simulink model "all_nn_0001_0127"  (R2026a)
settings: Solver=ode45  StopTime=40  AbsTol=1e-6
undefined symbols (not defined in the file): u_ts
settings Model: ExtModeTrigMode=oneshot  ExtModeArmWhenConnect=off  TunableVars=prueba  TunableVarsStorageClass=Auto  Creator=The MathWorks Inc.  LastModifiedBy=harry_31916
settings DataIOCC: SignalLoggingName=sigsOut
settings OptimizationCC: BooleanDataType=off  InitFltsAndDblsToZero=on
settings DebuggingCC: SaveWithParameterizedLinksMsg=none  UnderspecifiedInitializationDetection=Classic  SignalResolutionControl=TryResolveAllWithWarning  MultiTaskDSMMsg=warning  MultiTaskCondExecSysMsg=none
settings HardwareCC: ProdHWDeviceType=32-bit Generic  TargetUnknown=on
settings RTWCC: TemplateMakefile=grt_vc.tmf
settings GRTTargetCC: TargetFcnLib=ansi_tfl_tmw.mat  CombineOutputUpdateFcns=off  GRTInterface=on

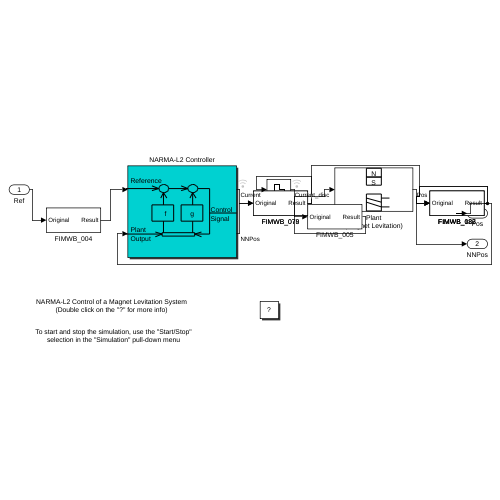
[thumbnail: Simulink's stored preview of the top-level diagram]
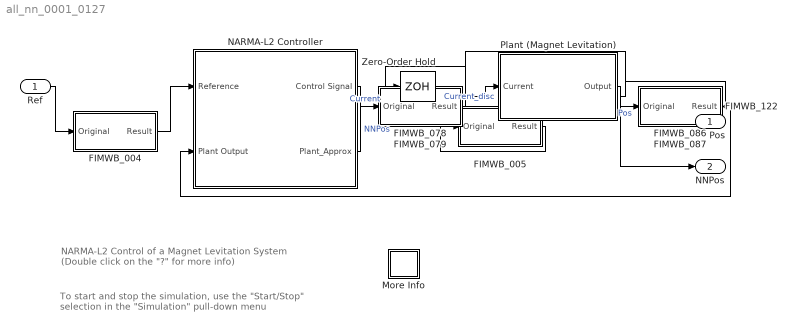
== system all_nn_0001_0127 ==
  note: NARMA-L2 Control of a Magnet Levitation System
      | (Double click on the "?" for more info)
  note: To start and stop the simulation, use the "Start/Stop"
      | selection in the "Simulation" pull-down menu
  Ref : Inport  Interpolate=off
  FIMWB_004 : Subsystem  Tag=fimwb.fault.4
  FIMWB_005 : Subsystem  Tag=fimwb.fault.5
  FIMWB_078 : Subsystem  Tag=fimwb.fault.78
  FIMWB_079 : Subsystem  Tag=fimwb.fault.79
  FIMWB_086 : Subsystem  Tag=fimwb.fault.86
  FIMWB_087 : Subsystem  Tag=fimwb.fault.87
  FIMWB_122 : Subsystem  Tag=fimwb.fault.122
  More Info : Subsystem
      mask Display: disp('?')
  NARMA-L2 Controller : Subsystem  mask(NARMA-L2 Controller){Ts=0.01, S1=9, Ni=3, Nj=2, sim_file=ballrepel0, trainfun=trainlm, Use_validation=1, Use_Testing=1, max_i=4, min_i=-1, max_i_int=1, min_i_int=0.1, sam_training=10000, epochs=100, minp=-0.97682887932966278033, maxp=3.9954019738068033973, mint=0.0012713472471279200528, maxt=3.9954019738068033973, Normalize=1, IW1_1=[2.8569160539166240653 3.855137973617931646 2.4478436741338867044 0.86889986713150191289;0.86019748624118552716 -0.76099748761653862594 0.12978383283599650988 -0.032681949683702651854;-0.61268951567451579443 -1.3546538767805089698 -1.0357145918607806312 -2.2450213565212968625;-0.61363639390594604262 3.6302797918127760468 -2.9742392265006136753 3.7505205510025696469;8.2159425419552984948 -0.34781842703357196411 -0.63990978222347083548 3.2203753164455033442;-0.55585558555235048406 1.7347260034225613357 -0.48782067399191109125 0.15519292550861990554;0.14490936608588075862 0.091344996887225110571 -1.9999177921909609967 -1.7398058021589537514;-0.011364174849476511159 0.17210174153872684344 -0.063003341331735851494 0.016356680939399299846;1.9115353490253352842 -1.6928290742800000679 0.26139115964517828372 -0.083521590880859600259], IW3_2=[2.094012153469472004 4.1391617494602943594 0.46017743638858904509 1.4212453617040687881;-0.8698291152927356551 -0.91216393263270156844 -1.7725276755524563832 -1.8256681774546807961;-1.5212626080129232342 -1.9638393468584769419 -0.13083206166844379981 0.69514443101461376173;1.1067100747068669975 1.1077222299712199405 -1.6499992245985941608 -0.10283142888325141895;1.7627456897433946281 0.12387727106338465577 -0.74345872574560734058 1.3295242695796243293;1.3902623706994512442 1.2486843128494045096 0.60100357220348832321 1.8703374952532536568;-1.2652620294004319756 -0.81003971518970829813 0.35904126229892613376 -2.3590512744589045013;-1.7962091138833455872 0.33004248956449860897 1.1996735804361835509 -0.75846441756669458201;1.6085665816521634852 -0.65960011993077061199 2.0409314507416924656 1.300834198719902135], IW5_3=-0.86130216008060445088, LW2_1=[5.755548244449743792e-05 2.1941017287714528194 -0.00044492281828180146918 -0.00039237971120205448854 1.8234323877817898572e-06 0.042708432151687514278 0.00025330049100551882673 4.7927194580095164866 0.41991364122019325666], LW4_3=[1.1796229157074380467 1.4349048600431937306 -0.8972572979998952869 -2.3386270416842869224 -0.096692942439327439486 -0.63438599215078772531 -2.7379194644695021843 3.0145214892072624835 2.1741978843496214679], LW5_4=0.59967978592905768487, LW6_5=0.00041169382628446888304, LW6_2=0.99216750753278892816, B1=[-2.0540485030510766684;-0.2820456548276839559;-1.4224984046874724619;0.011980000365264734455;-3.2833055176157808219;1.1020848049883287256;2.2616940700361274352;-0.14165422591960777354;1.0889769241125049071], B2=0.90790507647934137747, B3=[-0.99822473976112757743;-1.1258457923320430716;1.0030562696131117839;3.6020655513043440266;-0.0251859643674823587;1.2763936285299730677;-2.2740100652873409537;-3.0720977283302817185;1.7835104510380932474], B4=0.8636776698074994929, Limit_output=1, min_output=0, max_output=Inf, Use_Previous_Weights=1}
      mask prompts: Ts "Sample time"; trainfun "Training function"
      mask help: NARMA-L2 Controller. You first train a neural network model of the plant to be controlled. The controller is a rearrangement of the trained plant model. Double-click the NARMA-L2 Controller block to begin the plant training.
      mask init:
      | xl = [0    .4   NaN  .33  .55   .55  .33  .33  NaN .80  .92 .92];
      | yl = [.95 .95 NaN  .75  .75   .55  .55  .75  NaN  .95 .95 .65];
      | x2 = [0    .43 NaN .45 .45    NaN .92 1.2 NaN .63 .85 .85 .63 .63 ];
      | y2 = [.39 .39 NaN  .41 .55   NaN .65 .65 NaN .75 .75  .55  .55  .75];
      | x3 = [.45 .45 NaN .42 .45 .48  NaN .33 .4 .33];
      | y3 = [.75 .90 NaN .83 .90 .83  NaN  .98 .95 .92];
      | x4 = [.75 .75 NaN .72 .75 .78  NaN  .5 .7 NaN .63 .7 .63];
      | y4 = [.75 .90 NaN .83 .90 .83  NaN .95 .95 NaN .98 .95 .92];
      | x5 = [.43 .43 .77 .77 .43 NaN .36 .43 .36 NaN .75 .75];
      | y5 = [.37 .41 .41 .37 .37 NaN .42 .39 .36 NaN .41 .55];
      | x6 = [.92 .92 .77 NaN .84 .77 .84];
      | y6 = [.65 .39 .39 NaN .42 .39 .36];
      | x1t=.03; y1t=.31;
      | x2t=.03; y2t=.85;
      | x8t=.03;y8t=.21;
      | x3t=.77; y3t=.53;
      | x4t=.77; y4t=.44;
      | x5t=.34; y5t=.49;
      | x6t=.58; y6t=.49;
      | 
      | 
      | t=(0:24)/24*2*pi;
      | xs = .05*cos(t);
      | ys = .05*sin(t);
      | xs1=xs+.45;
      | ys1=ys+.95;
      | xs2=xs+.75;
      | ys2=ys+.95;
      settings: OpenFcn=nncontrolutil('nnident','',gcbh,gcb,'narma_l2');
      mask TypeOptions trainfun: trainbfg | trainbr  | traincgb | traincgf | traincgp | traingd | traingdm | traingda | traingdx | trainlm  | trainoss | trainrp  | trainscg
      mask Display:
      | plot([[xl NaN x2]*.9-.075 ], [[yl  NaN y2]*.9-.1 ]);
      | plot([[x3 NaN xs1 NaN xs2]*.9-.075 ], [[y3 NaN ys1 NaN ys2]*.9-.1 ]);
      | plot([x4 NaN x5]*.9-.075,[y4 NaN y5]*.9-.1);
      | plot([x6 NaN ]*.9-.075,[y6 NaN ]*.9-.1);
      | text(x1t,y1t,'Plant');
      | text(x8t,y8t,'Output');
      | text(x2t,y2t,'Reference');
      | text(x3t,y3t,'Control');
      | text(x4t,y4t,'Signal');
      | text(x5t,y5t,'f');
      | text(x6t,y6t,'g');
  Plant (Magnet Levitation) : Subsystem
      mask init:
      | x1=[-2 -2 2 2 -2 NaN -2 -2 2 2 -2];
      | y1=[5 4 4 5 5 NaN 2 0 0 2 2];
      | x2=[-2 -2 2 2 -2 NaN -2   2  NaN -2 2 NaN 2    4    NaN 2  4];
      | y2=[4  3  3 4  4 NaN 1.5 1  NaN 1 .5 NaN 1.5 1.5 NaN .5 .5];
      | x1t = -.5 ; y1t = 4.4;
      | x2t = -.5; y2t = 3.4;
      mask Display:
      | plot([-10],[0],[10],[5]);
      | plot([x1 NaN x2],[y1 NaN y2]);
      | text(x1t,y1t,'N')
      | text(x2t,y2t,'S')
  Zero-Order Hold : ZeroOrderHold  SampleTime=u_ts
  Pos : Outport  VectorParamsAs1DForOutWhenUnconnected=off
  NNPos : Outport  Port=2  VectorParamsAs1DForOutWhenUnconnected=off
  wires:
  Plant (Magnet Levitation)/1(Output) -> FIMWB_122/1(Original)  "Pos"
  FIMWB_122/1(Result) -> FIMWB_086/1(Original), FIMWB_087/1(Original)
  Ref/1 -> FIMWB_004/1(Original)
  FIMWB_004/1(Result) -> NARMA-L2 Controller/1(Reference)
  Zero-Order Hold/1 -> FIMWB_005/1(Original)  "Current_disc"
  FIMWB_005/1(Result) -> Plant (Magnet Levitation)/1(Current)
  NARMA-L2 Controller/1(Control Signal) -> FIMWB_078/1(Original)  "Current"
  FIMWB_078/1(Result) -> Zero-Order Hold/1
  NARMA-L2 Controller/2(Plant_Approx) -> FIMWB_079/1(Original)  "NNPos"
  FIMWB_079/1(Result) -> NNPos/1
  FIMWB_086/1(Result) -> Pos/1
  FIMWB_087/1(Result) -> NARMA-L2 Controller/2(Plant Output)

== system all_nn_0001_0127/FIMWB_004 ==
  Original : Inport
  Result : Outport
  wires:
  Original/1 -> Result/1

== system all_nn_0001_0127/FIMWB_005 ==
  Original : Inport
  Result : Outport
  wires:
  Original/1 -> Result/1

== system all_nn_0001_0127/FIMWB_078 ==
  Original : Inport
  Result : Outport
  wires:
  Original/1 -> Result/1

== system all_nn_0001_0127/FIMWB_079 ==
  Original : Inport
  Result : Outport
  wires:
  Original/1 -> Result/1

== system all_nn_0001_0127/FIMWB_086 ==
  Original : Inport
  Result : Outport
  wires:
  Original/1 -> Result/1

== system all_nn_0001_0127/FIMWB_087 ==
  Original : Inport
  Result : Outport
  wires:
  Original/1 -> Result/1

== system all_nn_0001_0127/FIMWB_122 ==
  Original : Inport
  Result : Outport
  wires:
  Original/1 -> Result/1

== system all_nn_0001_0127/More Info ==
  note: This system simulates NARMA-L2 control
      | of a magnet suspended by an electromagnet.
  note: Double-click on the NARMA-L2 Controller block
      | to train the neural network controller and plant model.
  note: For more information on what the controller
      | does, look under the mask of the NARMA-L2
      | Controller block.

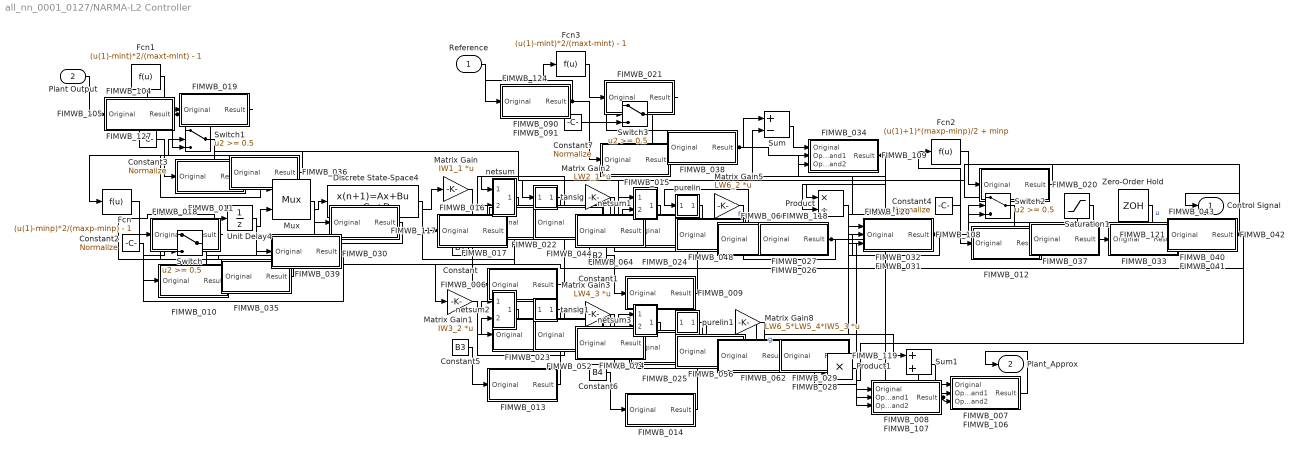
== system all_nn_0001_0127/NARMA-L2 Controller ==
  Reference : Inport
  Plant Output : Inport  Port=2
  Constant : Constant  Value=B1
  Constant1 : Constant  Value=B2
  Constant{2..4,7} (4 alike) : Constant  Value=Normalize
  Constant5 : Constant  Value=B3
  Constant6 : Constant  Value=B4
  Discrete State-Space4 : DiscreteStateSpace  A=blkdiag([zeros(1,Nj-1);eye(Nj-2,Nj-2) zeros(Nj-2,1)],[zeros(1,Ni-1);eye(Ni-2,Ni-2) zeros(Ni-2,1)])  B=blkdiag(eye(Nj-1,1),eye(Ni-1,1))  C=blkdiag([zeros(1,Nj-1);eye(Nj-1,Nj-1)],[zeros(eye(double(Ni>1)),Ni-1);eye(Ni-2,Ni-1)])  D=blkdiag([1;zeros(Nj-1,1)],[eye(double(Ni>1));zeros(Ni-2,1)])  SampleTime=Ts
  FIMWB_006 : Subsystem  Tag=fimwb.fault.6
  FIMWB_007 : Subsystem  Tag=fimwb.fault.7
  FIMWB_008 : Subsystem  Tag=fimwb.fault.8
  FIMWB_009 : Subsystem  Tag=fimwb.fault.9
  FIMWB_010 : Subsystem  Tag=fimwb.fault.10
  FIMWB_011 : Subsystem  Tag=fimwb.fault.11
  FIMWB_012 : Subsystem  Tag=fimwb.fault.12
  FIMWB_013 : Subsystem  Tag=fimwb.fault.13
  FIMWB_014 : Subsystem  Tag=fimwb.fault.14
  FIMWB_015 : Subsystem  Tag=fimwb.fault.15
  FIMWB_016 : Subsystem  Tag=fimwb.fault.16
  FIMWB_017 : Subsystem  Tag=fimwb.fault.17
  FIMWB_018 : Subsystem  Tag=fimwb.fault.18
  FIMWB_019 : Subsystem  Tag=fimwb.fault.19
  FIMWB_020 : Subsystem  Tag=fimwb.fault.20
  FIMWB_021 : Subsystem  Tag=fimwb.fault.21
  FIMWB_022 : Subsystem  Tag=fimwb.fault.22
  FIMWB_023 : Subsystem  Tag=fimwb.fault.23
  FIMWB_024 : Subsystem  Tag=fimwb.fault.24
  FIMWB_025 : Subsystem  Tag=fimwb.fault.25
  FIMWB_026 : Subsystem  Tag=fimwb.fault.26
  FIMWB_027 : Subsystem  Tag=fimwb.fault.27
  FIMWB_028 : Subsystem  Tag=fimwb.fault.28
  FIMWB_029 : Subsystem  Tag=fimwb.fault.29
  FIMWB_030 : Subsystem  Tag=fimwb.fault.30
  FIMWB_031 : Subsystem  Tag=fimwb.fault.31
  FIMWB_032 : Subsystem  Tag=fimwb.fault.32
  FIMWB_033 : Subsystem  Tag=fimwb.fault.33
  FIMWB_034 : Subsystem  Tag=fimwb.fault.34
  FIMWB_035 : Subsystem  Tag=fimwb.fault.35
  FIMWB_036 : Subsystem  Tag=fimwb.fault.36
  FIMWB_037 : Subsystem  Tag=fimwb.fault.37
  FIMWB_038 : Subsystem  Tag=fimwb.fault.38
  FIMWB_039 : Subsystem  Tag=fimwb.fault.39
  FIMWB_040 : Subsystem  Tag=fimwb.fault.40
  FIMWB_041 : Subsystem  Tag=fimwb.fault.41
  FIMWB_042 : Subsystem  Tag=fimwb.fault.42
  FIMWB_043 : Subsystem  Tag=fimwb.fault.43
  FIMWB_044 : Subsystem  Tag=fimwb.fault.44
  FIMWB_048 : Subsystem  Tag=fimwb.fault.48
  FIMWB_052 : Subsystem  Tag=fimwb.fault.52
  FIMWB_056 : Subsystem  Tag=fimwb.fault.56
  FIMWB_060 : Subsystem  Tag=fimwb.fault.60
  FIMWB_062 : Subsystem  Tag=fimwb.fault.62
  FIMWB_064 : Subsystem  Tag=fimwb.fault.64
  FIMWB_074 : Subsystem  Tag=fimwb.fault.74
  FIMWB_090 : Subsystem  Tag=fimwb.fault.90
  FIMWB_091 : Subsystem  Tag=fimwb.fault.91
  FIMWB_104 : Subsystem  Tag=fimwb.fault.104
  FIMWB_105 : Subsystem  Tag=fimwb.fault.105
  FIMWB_106 : Subsystem  Tag=fimwb.fault.106
  FIMWB_107 : Subsystem  Tag=fimwb.fault.107
  FIMWB_108 : Subsystem  Tag=fimwb.fault.108
  FIMWB_109 : Subsystem  Tag=fimwb.fault.109
  FIMWB_117 : Subsystem  Tag=fimwb.fault.117
  FIMWB_118 : Subsystem  Tag=fimwb.fault.118
  FIMWB_119 : Subsystem  Tag=fimwb.fault.119
  FIMWB_120 : Subsystem  Tag=fimwb.fault.120
  FIMWB_121 : Subsystem  Tag=fimwb.fault.121
  FIMWB_124 : Subsystem  Tag=fimwb.fault.124
  FIMWB_127 : Subsystem  Tag=fimwb.fault.127
  Fcn : Fcn  Expr=(u(1)-minp)*2/(maxp-minp) - 1
  Fcn1 : Fcn  Expr=(u(1)-mint)*2/(maxt-mint) - 1
  Fcn2 : Fcn  Expr=(u(1)+1)*(maxp-minp)/2 + minp
  Fcn3 : Fcn  Expr=(u(1)-mint)*2/(maxt-mint) - 1
  Matrix Gain : Gain  Gain=IW1_1  Multiplication=Matrix(K*u)  SaturateOnIntegerOverflow=on  OutDataTypeStr=Inherit: Same as input  ParamDataTypeStr=Inherit: Same as input
  Matrix Gain1 : Gain  Gain=IW3_2  Multiplication=Matrix(K*u)  SaturateOnIntegerOverflow=on  OutDataTypeStr=Inherit: Same as input  ParamDataTypeStr=Inherit: Same as input
  Matrix Gain2 : Gain  Gain=LW2_1  Multiplication=Matrix(K*u)  SaturateOnIntegerOverflow=on  OutDataTypeStr=Inherit: Same as input  ParamDataTypeStr=Inherit: Same as input
  Matrix Gain3 : Gain  Gain=LW4_3  Multiplication=Matrix(K*u)  SaturateOnIntegerOverflow=on  OutDataTypeStr=Inherit: Same as input  ParamDataTypeStr=Inherit: Same as input
  Matrix Gain5 : Gain  Gain=LW6_2  Multiplication=Matrix(K*u)  SaturateOnIntegerOverflow=on  OutDataTypeStr=Inherit: Same as input  ParamDataTypeStr=Inherit: Same as input
  Matrix Gain8 : Gain  Gain=LW6_5*LW5_4*IW5_3  Multiplication=Matrix(K*u)  SaturateOnIntegerOverflow=on  OutDataTypeStr=Inherit: Same as input  ParamDataTypeStr=Inherit: Same as input
  Mux : Mux  Inputs=2
      settings: DisplayOption=signals
  Product : Product  Inputs=*/  InputSameDT=on  SaturateOnIntegerOverflow=on  OutDataTypeStr=Inherit: Same as first input
  Product1 : Product  InputSameDT=on  SaturateOnIntegerOverflow=on  OutDataTypeStr=Inherit: Same as first input
  Saturation1 : Saturate  UpperLimit=max_i  LowerLimit=min_i  ZeroCross=off
  Sum : Sum  Inputs=+-  InputSameDT=on  SaturateOnIntegerOverflow=on  OutDataTypeStr=Inherit: Same as first input
  Sum1 : Sum  InputSameDT=on  SaturateOnIntegerOverflow=on  OutDataTypeStr=Inherit: Same as first input
  Switch{,1..3} (4 alike) : Switch  Threshold=0.5  ZeroCross=off
  Unit Delay4 : UnitDelay  SampleTime=Ts
  Zero-Order Hold : ZeroOrderHold  SampleTime=Ts
  netsum : Subsystem
      mask Display: disp('+')
  netsum1 : Subsystem
      mask Display: disp('+')
  netsum2 : Subsystem
      mask Display: disp('+')
  netsum3 : Subsystem
      mask Display: disp('+')
  purelin : Subsystem
      mask Display: plot([-1 1],[0 0],[-1 1],[-1 1])
  purelin1 : Subsystem
      mask Display: plot([-1 1],[0 0],[-1 1],[-1 1])
  tansig : Subsystem
      mask Display: plot([-1 1],[0 0],[-1 -.9 -.8 -.7 -.6 -.5 -.4 -.3 -.2 -.1 0 .1 .2 .3 .4 .5 .6 .7 .8 .9 1],2./(1+exp(-8*[-1 -.9 -.8 -.7 -.6 -.5 -.4 -.3 -.2 -.1 0 .1 .2 .3 .4 .5 .6 .7 .8 .9 1]))-1)
  tansig1 : Subsystem
      mask Display: plot([-1 1],[0 0],[-1 -.9 -.8 -.7 -.6 -.5 -.4 -.3 -.2 -.1 0 .1 .2 .3 .4 .5 .6 .7 .8 .9 1],2./(1+exp(-8*[-1 -.9 -.8 -.7 -.6 -.5 -.4 -.3 -.2 -.1 0 .1 .2 .3 .4 .5 .6 .7 .8 .9 1]))-1)
  Control Signal : Outport  VectorParamsAs1DForOutWhenUnconnected=off
  Plant_Approx : Outport  Port=2  VectorParamsAs1DForOutWhenUnconnected=off
  wires:
  Sum1/1 -> FIMWB_106/1(Original)
  Product1/1 -> FIMWB_107/1(Original)
  Product/1 -> FIMWB_108/1(Original)
  Sum/1 -> FIMWB_109/1(Original)
  Discrete State-Space4/1 -> FIMWB_117/1(Original)
  FIMWB_117/1(Result) -> FIMWB_016/1(Original), FIMWB_017/1(Original)
  Matrix Gain5/1 -> FIMWB_118/1(Original)  "f"
  FIMWB_118/1(Result) -> FIMWB_026/1(Original), FIMWB_027/1(Original)
  Matrix Gain8/1 -> FIMWB_119/1(Original)  "g"
  FIMWB_119/1(Result) -> FIMWB_028/1(Original), FIMWB_029/1(Original)
  FIMWB_108/1(Result) -> FIMWB_120/1(Original)
  FIMWB_120/1(Result) -> FIMWB_031/1(Original), FIMWB_032/1(Original)
  Zero-Order Hold/1 -> FIMWB_121/1(Original)  "u"
  FIMWB_121/1(Result) -> FIMWB_040/1(Original), FIMWB_041/1(Original), FIMWB_042/1(Original), FIMWB_043/1(Original)
  Reference/1 -> FIMWB_124/1(Original)
  FIMWB_124/1(Result) -> FIMWB_090/1(Original), FIMWB_091/1(Original)
  Plant Output/1 -> FIMWB_127/1(Original)
  FIMWB_127/1(Result) -> FIMWB_104/1(Original), FIMWB_105/1(Original)
  Constant/1 -> FIMWB_006/1(Original)
  FIMWB_006/1(Result) -> netsum/2(In2)
  FIMWB_106/1(Result) -> FIMWB_007/1(Original)
  FIMWB_007/1(Result) -> Plant_Approx/1
  FIMWB_107/1(Result) -> FIMWB_008/1(Original)
  FIMWB_008/1(Result) -> Sum1/2, FIMWB_106/3(Operand2)
  Constant1/1 -> FIMWB_009/1(Original)
  FIMWB_009/1(Result) -> netsum1/2(In2)
  Constant2/1 -> FIMWB_010/1(Original)
  FIMWB_010/1(Result) -> Switch/2
  Constant3/1 -> FIMWB_011/1(Original)
  FIMWB_011/1(Result) -> Switch1/2
  Constant4/1 -> FIMWB_012/1(Original)
  FIMWB_012/1(Result) -> Switch2/2
  Constant5/1 -> FIMWB_013/1(Original)
  FIMWB_013/1(Result) -> netsum2/2(In2)
  Constant6/1 -> FIMWB_014/1(Original)
  FIMWB_014/1(Result) -> netsum3/2(In2)
  Constant7/1 -> FIMWB_015/1(Original)
  FIMWB_015/1(Result) -> Switch3/2
  FIMWB_016/1(Result) -> Matrix Gain/1
  FIMWB_017/1(Result) -> Matrix Gain1/1
  Fcn/1 -> FIMWB_018/1(Original)
  FIMWB_018/1(Result) -> Switch/1
  Fcn1/1 -> FIMWB_019/1(Original)
  FIMWB_019/1(Result) -> Switch1/1
  Fcn2/1 -> FIMWB_020/1(Original)
  FIMWB_020/1(Result) -> Switch2/1
  Fcn3/1 -> FIMWB_021/1(Original)
  FIMWB_021/1(Result) -> Switch3/1
  Matrix Gain/1 -> FIMWB_022/1(Original)
  FIMWB_022/1(Result) -> netsum/1(In1)
  Matrix Gain1/1 -> FIMWB_023/1(Original)
  FIMWB_023/1(Result) -> netsum2/1(In1)
  Matrix Gain2/1 -> FIMWB_024/1(Original)
  FIMWB_024/1(Result) -> netsum1/1(In1)
  Matrix Gain3/1 -> FIMWB_025/1(Original)
  FIMWB_025/1(Result) -> netsum3/1(In1)
  FIMWB_026/1(Result) -> Sum1/1, FIMWB_106/2(Operand1)
  FIMWB_027/1(Result) -> Sum/2, FIMWB_109/3(Operand2)
  FIMWB_028/1(Result) -> Product1/1, FIMWB_107/2(Operand1)
  FIMWB_029/1(Result) -> Product/2, FIMWB_108/3(Operand2)
  Mux/1 -> FIMWB_030/1(Original)
  FIMWB_030/1(Result) -> Discrete State-Space4/1
  FIMWB_031/1(Result) -> Fcn2/1
  FIMWB_032/1(Result) -> Switch2/3
  Saturation1/1 -> FIMWB_033/1(Original)
  FIMWB_033/1(Result) -> Zero-Order Hold/1
  FIMWB_109/1(Result) -> FIMWB_034/1(Original)
  FIMWB_034/1(Result) -> Product/1, FIMWB_108/2(Operand1)
  Switch/1 -> FIMWB_035/1(Original)
  FIMWB_035/1(Result) -> Unit Delay4/1
  Switch1/1 -> FIMWB_036/1(Original)
  FIMWB_036/1(Result) -> Mux/1
  Switch2/1 -> FIMWB_037/1(Original)
  FIMWB_037/1(Result) -> Saturation1/1
  Switch3/1 -> FIMWB_038/1(Original)
  FIMWB_038/1(Result) -> Sum/1, FIMWB_109/2(Operand1)
  Unit Delay4/1 -> FIMWB_039/1(Original)
  FIMWB_039/1(Result) -> Mux/2
  FIMWB_040/1(Result) -> Product1/2, FIMWB_107/3(Operand2)
  FIMWB_041/1(Result) -> Fcn/1
  FIMWB_042/1(Result) -> Switch/3
  FIMWB_043/1(Result) -> Control Signal/1
  netsum/1(Out1) -> FIMWB_044/1(Original)
  FIMWB_044/1(Result) -> tansig/1(n)
  netsum1/1(Out1) -> FIMWB_048/1(Original)
  FIMWB_048/1(Result) -> purelin/1(n)
  netsum2/1(Out1) -> FIMWB_052/1(Original)
  FIMWB_052/1(Result) -> tansig1/1(n)
  netsum3/1(Out1) -> FIMWB_056/1(Original)
  FIMWB_056/1(Result) -> purelin1/1(n)
  purelin/1(a) -> FIMWB_060/1(Original)
  FIMWB_060/1(Result) -> Matrix Gain5/1
  purelin1/1(a) -> FIMWB_062/1(Original)
  FIMWB_062/1(Result) -> Matrix Gain8/1
  tansig/1(a) -> FIMWB_064/1(Original)
  FIMWB_064/1(Result) -> Matrix Gain2/1
  tansig1/1(a) -> FIMWB_074/1(Original)
  FIMWB_074/1(Result) -> Matrix Gain3/1
  FIMWB_090/1(Result) -> Fcn3/1
  FIMWB_091/1(Result) -> Switch3/3
  FIMWB_104/1(Result) -> Fcn1/1
  FIMWB_105/1(Result) -> Switch1/3

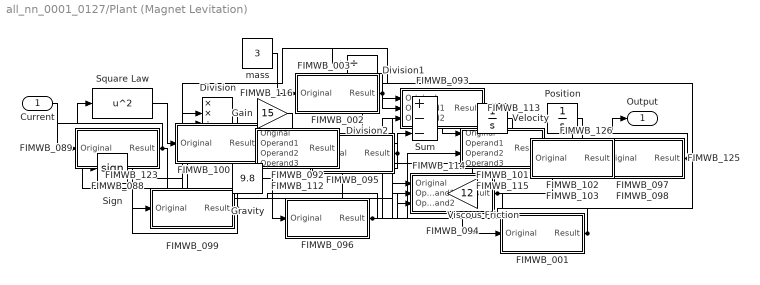
== system all_nn_0001_0127/Plant (Magnet Levitation) ==
  Current : Inport
  Division : Product  Inputs=**/  InputSameDT=on  SaturateOnIntegerOverflow=on  OutDataTypeStr=Inherit: Same as first input
  Division1 : Product  Inputs=/*  InputSameDT=on  SaturateOnIntegerOverflow=on  OutDataTypeStr=Inherit: Same as first input
  Division2 : Product  Inputs=/*  InputSameDT=on  SaturateOnIntegerOverflow=on  OutDataTypeStr=Inherit: Same as first input
  FIMWB_001 : Subsystem  Tag=fimwb.fault.1
  FIMWB_002 : Subsystem  Tag=fimwb.fault.2
  FIMWB_003 : Subsystem  Tag=fimwb.fault.3
  FIMWB_088 : Subsystem  Tag=fimwb.fault.88
  FIMWB_089 : Subsystem  Tag=fimwb.fault.89
  FIMWB_092 : Subsystem  Tag=fimwb.fault.92
  FIMWB_093 : Subsystem  Tag=fimwb.fault.93
  FIMWB_094 : Subsystem  Tag=fimwb.fault.94
  FIMWB_095 : Subsystem  Tag=fimwb.fault.95
  FIMWB_096 : Subsystem  Tag=fimwb.fault.96
  FIMWB_097 : Subsystem  Tag=fimwb.fault.97
  FIMWB_098 : Subsystem  Tag=fimwb.fault.98
  FIMWB_099 : Subsystem  Tag=fimwb.fault.99
  FIMWB_100 : Subsystem  Tag=fimwb.fault.100
  FIMWB_101 : Subsystem  Tag=fimwb.fault.101
  FIMWB_102 : Subsystem  Tag=fimwb.fault.102
  FIMWB_103 : Subsystem  Tag=fimwb.fault.103
  FIMWB_112 : Subsystem  Tag=fimwb.fault.112
  FIMWB_113 : Subsystem  Tag=fimwb.fault.113
  FIMWB_114 : Subsystem  Tag=fimwb.fault.114
  FIMWB_115 : Subsystem  Tag=fimwb.fault.115
  FIMWB_116 : Subsystem  Tag=fimwb.fault.116
  FIMWB_123 : Subsystem  Tag=fimwb.fault.123
  FIMWB_125 : Subsystem  Tag=fimwb.fault.125
  FIMWB_126 : Subsystem  Tag=fimwb.fault.126
  Gain : Gain  Gain=15  SaturateOnIntegerOverflow=on  OutDataTypeStr=Inherit: Same as input  ParamDataTypeStr=Inherit: Same as input
  Gravity : Constant  Value=9.8
  Position : Integrator  InitialCondition=.5  ZeroCross=off
  Sign : Signum  ZeroCross=off
  Square Law : Fcn  Expr=u^2
  Sum : Sum  Inputs=|+--  InputSameDT=on  SaturateOnIntegerOverflow=on  OutDataTypeStr=Inherit: Same as first input
  Velocity : Integrator  ZeroCross=off
  Viscous Friction : Gain  Gain=12  SaturateOnIntegerOverflow=on  OutDataTypeStr=Inherit: Same as input  ParamDataTypeStr=Inherit: Same as input
  mass : Constant  Value=3
  Output : Outport  VectorParamsAs1DForOutWhenUnconnected=off
  wires:
  Division/1 -> FIMWB_112/1(Original)
  Division1/1 -> FIMWB_113/1(Original)
  Division2/1 -> FIMWB_114/1(Original)
  Sum/1 -> FIMWB_115/1(Original)
  mass/1 -> FIMWB_116/1(Original)
  FIMWB_116/1(Result) -> FIMWB_002/1(Original), FIMWB_003/1(Original)
  Current/1 -> FIMWB_123/1(Original)
  FIMWB_123/1(Result) -> FIMWB_088/1(Original), FIMWB_089/1(Original)
  Position/1 -> FIMWB_125/1(Original)
  FIMWB_125/1(Result) -> FIMWB_097/1(Original), FIMWB_098/1(Original)
  Velocity/1 -> FIMWB_126/1(Original)
  FIMWB_126/1(Result) -> FIMWB_102/1(Original), FIMWB_103/1(Original)
  Viscous Friction/1 -> FIMWB_001/1(Original)
  FIMWB_001/1(Result) -> Division2/2, FIMWB_114/3(Operand2)
  FIMWB_002/1(Result) -> Division1/1, FIMWB_113/2(Operand1)
  FIMWB_003/1(Result) -> Division2/1, FIMWB_114/2(Operand1)
  FIMWB_088/1(Result) -> Sign/1
  FIMWB_089/1(Result) -> Square Law/1
  FIMWB_112/1(Result) -> FIMWB_092/1(Original)
  FIMWB_092/1(Result) -> Gain/1
  FIMWB_113/1(Result) -> FIMWB_093/1(Original)
  FIMWB_093/1(Result) -> Sum/1, FIMWB_115/2(Operand1)
  FIMWB_114/1(Result) -> FIMWB_094/1(Original)
  FIMWB_094/1(Result) -> Sum/3, FIMWB_115/4(Operand3)
  Gain/1 -> FIMWB_095/1(Original)
  FIMWB_095/1(Result) -> Division1/2, FIMWB_113/3(Operand2)
  Gravity/1 -> FIMWB_096/1(Original)
  FIMWB_096/1(Result) -> Sum/2, FIMWB_115/3(Operand2)
  FIMWB_097/1(Result) -> Output/1
  FIMWB_098/1(Result) -> Division/3, FIMWB_112/4(Operand3)
  Sign/1 -> FIMWB_099/1(Original)
  FIMWB_099/1(Result) -> Division/2, FIMWB_112/3(Operand2)
  Square Law/1 -> FIMWB_100/1(Original)
  FIMWB_100/1(Result) -> Division/1, FIMWB_112/2(Operand1)
  FIMWB_115/1(Result) -> FIMWB_101/1(Original)
  FIMWB_101/1(Result) -> Velocity/1
  FIMWB_102/1(Result) -> Viscous Friction/1
  FIMWB_103/1(Result) -> Position/1

== system all_nn_0001_0127/NARMA-L2 Controller/FIMWB_006 ==
  Original : Inport
  Result : Outport
  wires:
  Original/1 -> Result/1

== system all_nn_0001_0127/NARMA-L2 Controller/FIMWB_007 ==
  Original : Inport
  Result : Outport
  wires:
  Original/1 -> Result/1

== system all_nn_0001_0127/NARMA-L2 Controller/FIMWB_008 ==
  Original : Inport
  Result : Outport
  wires:
  Original/1 -> Result/1

== system all_nn_0001_0127/NARMA-L2 Controller/FIMWB_009 ==
  Original : Inport
  Result : Outport
  wires:
  Original/1 -> Result/1

== system all_nn_0001_0127/NARMA-L2 Controller/FIMWB_010 ==
  Original : Inport
  Result : Outport
  wires:
  Original/1 -> Result/1

== system all_nn_0001_0127/NARMA-L2 Controller/FIMWB_011 ==
  Original : Inport
  Result : Outport
  wires:
  Original/1 -> Result/1

== system all_nn_0001_0127/NARMA-L2 Controller/FIMWB_012 ==
  Original : Inport
  Result : Outport
  wires:
  Original/1 -> Result/1

== system all_nn_0001_0127/NARMA-L2 Controller/FIMWB_013 ==
  Original : Inport
  Result : Outport
  wires:
  Original/1 -> Result/1

== system all_nn_0001_0127/NARMA-L2 Controller/FIMWB_014 ==
  Original : Inport
  Result : Outport
  wires:
  Original/1 -> Result/1

== system all_nn_0001_0127/NARMA-L2 Controller/FIMWB_015 ==
  Original : Inport
  Result : Outport
  wires:
  Original/1 -> Result/1

== system all_nn_0001_0127/NARMA-L2 Controller/FIMWB_016 ==
  Original : Inport
  Result : Outport
  wires:
  Original/1 -> Result/1

== system all_nn_0001_0127/NARMA-L2 Controller/FIMWB_017 ==
  Original : Inport
  Result : Outport
  wires:
  Original/1 -> Result/1

== system all_nn_0001_0127/NARMA-L2 Controller/FIMWB_018 ==
  Original : Inport
  Result : Outport
  wires:
  Original/1 -> Result/1

== system all_nn_0001_0127/NARMA-L2 Controller/FIMWB_019 ==
  Original : Inport
  Result : Outport
  wires:
  Original/1 -> Result/1

== system all_nn_0001_0127/NARMA-L2 Controller/FIMWB_020 ==
  Original : Inport
  Result : Outport
  wires:
  Original/1 -> Result/1

== system all_nn_0001_0127/NARMA-L2 Controller/FIMWB_021 ==
  Original : Inport
  Result : Outport
  wires:
  Original/1 -> Result/1

== system all_nn_0001_0127/NARMA-L2 Controller/FIMWB_022 ==
  Original : Inport
  Result : Outport
  wires:
  Original/1 -> Result/1

== system all_nn_0001_0127/NARMA-L2 Controller/FIMWB_023 ==
  Original : Inport
  Result : Outport
  wires:
  Original/1 -> Result/1

== system all_nn_0001_0127/NARMA-L2 Controller/FIMWB_024 ==
  Original : Inport
  Result : Outport
  wires:
  Original/1 -> Result/1

== system all_nn_0001_0127/NARMA-L2 Controller/FIMWB_025 ==
  Original : Inport
  Result : Outport
  wires:
  Original/1 -> Result/1

== system all_nn_0001_0127/NARMA-L2 Controller/FIMWB_026 ==
  Original : Inport
  Result : Outport
  wires:
  Original/1 -> Result/1

== system all_nn_0001_0127/NARMA-L2 Controller/FIMWB_027 ==
  Original : Inport
  Result : Outport
  wires:
  Original/1 -> Result/1

== system all_nn_0001_0127/NARMA-L2 Controller/FIMWB_028 ==
  Original : Inport
  Result : Outport
  wires:
  Original/1 -> Result/1

== system all_nn_0001_0127/NARMA-L2 Controller/FIMWB_029 ==
  Original : Inport
  Result : Outport
  wires:
  Original/1 -> Result/1

== system all_nn_0001_0127/NARMA-L2 Controller/FIMWB_030 ==
  Original : Inport
  Result : Outport
  wires:
  Original/1 -> Result/1

== system all_nn_0001_0127/NARMA-L2 Controller/FIMWB_031 ==
  Original : Inport
  Result : Outport
  wires:
  Original/1 -> Result/1

== system all_nn_0001_0127/NARMA-L2 Controller/FIMWB_032 ==
  Original : Inport
  Result : Outport
  wires:
  Original/1 -> Result/1

== system all_nn_0001_0127/NARMA-L2 Controller/FIMWB_033 ==
  Original : Inport
  Result : Outport
  wires:
  Original/1 -> Result/1

== system all_nn_0001_0127/NARMA-L2 Controller/FIMWB_034 ==
  Original : Inport
  Result : Outport
  wires:
  Original/1 -> Result/1

== system all_nn_0001_0127/NARMA-L2 Controller/FIMWB_035 ==
  Original : Inport
  Result : Outport
  wires:
  Original/1 -> Result/1

== system all_nn_0001_0127/NARMA-L2 Controller/FIMWB_036 ==
  Original : Inport
  Result : Outport
  wires:
  Original/1 -> Result/1

== system all_nn_0001_0127/NARMA-L2 Controller/FIMWB_037 ==
  Original : Inport
  Result : Outport
  wires:
  Original/1 -> Result/1

== system all_nn_0001_0127/NARMA-L2 Controller/FIMWB_038 ==
  Original : Inport
  Result : Outport
  wires:
  Original/1 -> Result/1

== system all_nn_0001_0127/NARMA-L2 Controller/FIMWB_039 ==
  Original : Inport
  Result : Outport
  wires:
  Original/1 -> Result/1

== system all_nn_0001_0127/NARMA-L2 Controller/FIMWB_040 ==
  Original : Inport
  Result : Outport
  wires:
  Original/1 -> Result/1

== system all_nn_0001_0127/NARMA-L2 Controller/FIMWB_041 ==
  Original : Inport
  Result : Outport
  wires:
  Original/1 -> Result/1

== system all_nn_0001_0127/NARMA-L2 Controller/FIMWB_042 ==
  Original : Inport
  Result : Outport
  wires:
  Original/1 -> Result/1

== system all_nn_0001_0127/NARMA-L2 Controller/FIMWB_043 ==
  Original : Inport
  Result : Outport
  wires:
  Original/1 -> Result/1

== system all_nn_0001_0127/NARMA-L2 Controller/FIMWB_044 ==
  Original : Inport
  Result : Outport
  wires:
  Original/1 -> Result/1

== system all_nn_0001_0127/NARMA-L2 Controller/FIMWB_048 ==
  Original : Inport
  Result : Outport
  wires:
  Original/1 -> Result/1

== system all_nn_0001_0127/NARMA-L2 Controller/FIMWB_052 ==
  Original : Inport
  Result : Outport
  wires:
  Original/1 -> Result/1

== system all_nn_0001_0127/NARMA-L2 Controller/FIMWB_056 ==
  Original : Inport
  Result : Outport
  wires:
  Original/1 -> Result/1

== system all_nn_0001_0127/NARMA-L2 Controller/FIMWB_060 ==
  Original : Inport
  Result : Outport
  wires:
  Original/1 -> Result/1

== system all_nn_0001_0127/NARMA-L2 Controller/FIMWB_062 ==
  Original : Inport
  Result : Outport
  wires:
  Original/1 -> Result/1

== system all_nn_0001_0127/NARMA-L2 Controller/FIMWB_064 ==
  Original : Inport
  Result : Outport
  wires:
  Original/1 -> Result/1

== system all_nn_0001_0127/NARMA-L2 Controller/FIMWB_074 ==
  Original : Inport
  Result : Outport
  wires:
  Original/1 -> Result/1

== system all_nn_0001_0127/NARMA-L2 Controller/FIMWB_090 ==
  Original : Inport
  Result : Outport
  wires:
  Original/1 -> Result/1

== system all_nn_0001_0127/NARMA-L2 Controller/FIMWB_091 ==
  Original : Inport
  Result : Outport
  wires:
  Original/1 -> Result/1

== system all_nn_0001_0127/NARMA-L2 Controller/FIMWB_104 ==
  Original : Inport
  Result : Outport
  wires:
  Original/1 -> Result/1

== system all_nn_0001_0127/NARMA-L2 Controller/FIMWB_105 ==
  Original : Inport
  Result : Outport
  wires:
  Original/1 -> Result/1

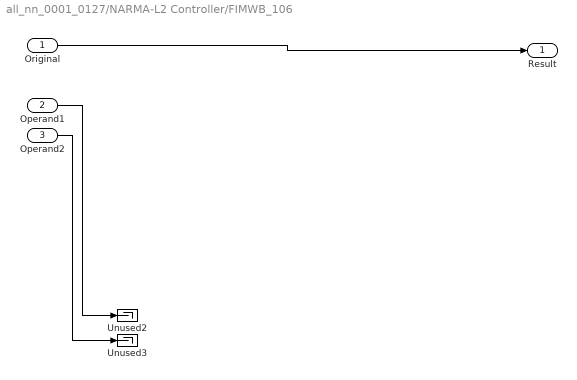
== system all_nn_0001_0127/NARMA-L2 Controller/FIMWB_106 ==
  Original : Inport
  Operand1 : Inport  Port=2
  Operand2 : Inport  Port=3
  Unused2 : Terminator
  Unused3 : Terminator
  Result : Outport
  wires:
  Original/1 -> Result/1
  Operand1/1 -> Unused2/1
  Operand2/1 -> Unused3/1

== system all_nn_0001_0127/NARMA-L2 Controller/FIMWB_107 ==
  Original : Inport
  Operand1 : Inport  Port=2
  Operand2 : Inport  Port=3
  Unused2 : Terminator
  Unused3 : Terminator
  Result : Outport
  wires:
  Original/1 -> Result/1
  Operand1/1 -> Unused2/1
  Operand2/1 -> Unused3/1

== system all_nn_0001_0127/NARMA-L2 Controller/FIMWB_108 ==
  Original : Inport
  Operand1 : Inport  Port=2
  Operand2 : Inport  Port=3
  Unused2 : Terminator
  Unused3 : Terminator
  Result : Outport
  wires:
  Original/1 -> Result/1
  Operand1/1 -> Unused2/1
  Operand2/1 -> Unused3/1

== system all_nn_0001_0127/NARMA-L2 Controller/FIMWB_109 ==
  Original : Inport
  Operand1 : Inport  Port=2
  Operand2 : Inport  Port=3
  Unused2 : Terminator
  Unused3 : Terminator
  Result : Outport
  wires:
  Original/1 -> Result/1
  Operand1/1 -> Unused2/1
  Operand2/1 -> Unused3/1

== system all_nn_0001_0127/NARMA-L2 Controller/FIMWB_117 ==
  Original : Inport
  Result : Outport
  wires:
  Original/1 -> Result/1

== system all_nn_0001_0127/NARMA-L2 Controller/FIMWB_118 ==
  Original : Inport
  Result : Outport
  wires:
  Original/1 -> Result/1

== system all_nn_0001_0127/NARMA-L2 Controller/FIMWB_119 ==
  Original : Inport
  Result : Outport
  wires:
  Original/1 -> Result/1

== system all_nn_0001_0127/NARMA-L2 Controller/FIMWB_120 ==
  Original : Inport
  Result : Outport
  wires:
  Original/1 -> Result/1

== system all_nn_0001_0127/NARMA-L2 Controller/FIMWB_121 ==
  Original : Inport
  Result : Outport
  wires:
  Original/1 -> Result/1

== system all_nn_0001_0127/NARMA-L2 Controller/FIMWB_124 ==
  Original : Inport
  Result : Outport
  wires:
  Original/1 -> Result/1

== system all_nn_0001_0127/NARMA-L2 Controller/FIMWB_127 ==
  Original : Inport
  Result : Outport
  wires:
  Original/1 -> Result/1

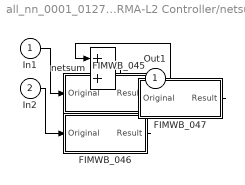
== system all_nn_0001_0127/NARMA-L2 Controller/netsum ==
  In1 : Inport
  In2 : Inport  Port=2
  FIMWB_045 : Subsystem  Tag=fimwb.fault.45
  FIMWB_046 : Subsystem  Tag=fimwb.fault.46
  FIMWB_047 : Subsystem  Tag=fimwb.fault.47
  netsum : Sum  Inputs=2  InputSameDT=on  SaturateOnIntegerOverflow=on  OutDataTypeStr=Inherit: Same as first input
  Out1 : Outport  VectorParamsAs1DForOutWhenUnconnected=off
  wires:
  In1/1 -> FIMWB_045/1(Original)
  FIMWB_045/1(Result) -> netsum/1
  In2/1 -> FIMWB_046/1(Original)
  FIMWB_046/1(Result) -> netsum/2
  netsum/1 -> FIMWB_047/1(Original)
  FIMWB_047/1(Result) -> Out1/1

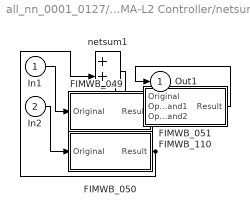
== system all_nn_0001_0127/NARMA-L2 Controller/netsum1 ==
  In1 : Inport
  In2 : Inport  Port=2
  FIMWB_049 : Subsystem  Tag=fimwb.fault.49
  FIMWB_050 : Subsystem  Tag=fimwb.fault.50
  FIMWB_051 : Subsystem  Tag=fimwb.fault.51
  FIMWB_110 : Subsystem  Tag=fimwb.fault.110
  netsum1 : Sum  Inputs=2  InputSameDT=on  SaturateOnIntegerOverflow=on  OutDataTypeStr=Inherit: Same as first input
  Out1 : Outport  VectorParamsAs1DForOutWhenUnconnected=off
  wires:
  netsum1/1 -> FIMWB_110/1(Original)
  In1/1 -> FIMWB_049/1(Original)
  FIMWB_049/1(Result) -> netsum1/1, FIMWB_110/2(Operand1)
  In2/1 -> FIMWB_050/1(Original)
  FIMWB_050/1(Result) -> netsum1/2, FIMWB_110/3(Operand2)
  FIMWB_110/1(Result) -> FIMWB_051/1(Original)
  FIMWB_051/1(Result) -> Out1/1

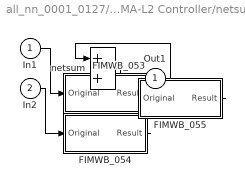
== system all_nn_0001_0127/NARMA-L2 Controller/netsum2 ==
  In1 : Inport
  In2 : Inport  Port=2
  FIMWB_053 : Subsystem  Tag=fimwb.fault.53
  FIMWB_054 : Subsystem  Tag=fimwb.fault.54
  FIMWB_055 : Subsystem  Tag=fimwb.fault.55
  netsum : Sum  Inputs=2  InputSameDT=on  SaturateOnIntegerOverflow=on  OutDataTypeStr=Inherit: Same as first input
  Out1 : Outport  VectorParamsAs1DForOutWhenUnconnected=off
  wires:
  In1/1 -> FIMWB_053/1(Original)
  FIMWB_053/1(Result) -> netsum/1
  In2/1 -> FIMWB_054/1(Original)
  FIMWB_054/1(Result) -> netsum/2
  netsum/1 -> FIMWB_055/1(Original)
  FIMWB_055/1(Result) -> Out1/1

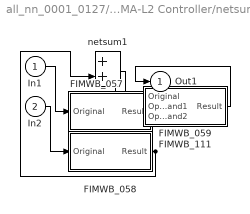
== system all_nn_0001_0127/NARMA-L2 Controller/netsum3 ==
  In1 : Inport
  In2 : Inport  Port=2
  FIMWB_057 : Subsystem  Tag=fimwb.fault.57
  FIMWB_058 : Subsystem  Tag=fimwb.fault.58
  FIMWB_059 : Subsystem  Tag=fimwb.fault.59
  FIMWB_111 : Subsystem  Tag=fimwb.fault.111
  netsum1 : Sum  Inputs=2  InputSameDT=on  SaturateOnIntegerOverflow=on  OutDataTypeStr=Inherit: Same as first input
  Out1 : Outport  VectorParamsAs1DForOutWhenUnconnected=off
  wires:
  netsum1/1 -> FIMWB_111/1(Original)
  In1/1 -> FIMWB_057/1(Original)
  FIMWB_057/1(Result) -> netsum1/1, FIMWB_111/2(Operand1)
  In2/1 -> FIMWB_058/1(Original)
  FIMWB_058/1(Result) -> netsum1/2, FIMWB_111/3(Operand2)
  FIMWB_111/1(Result) -> FIMWB_059/1(Original)
  FIMWB_059/1(Result) -> Out1/1

== system all_nn_0001_0127/NARMA-L2 Controller/purelin ==
  n : Inport
  FIMWB_061 : Subsystem  Tag=fimwb.fault.61
  a : Outport  VectorParamsAs1DForOutWhenUnconnected=off
  wires:
  n/1 -> FIMWB_061/1(Original)
  FIMWB_061/1(Result) -> a/1

== system all_nn_0001_0127/NARMA-L2 Controller/purelin1 ==
  n : Inport
  FIMWB_063 : Subsystem  Tag=fimwb.fault.63
  a : Outport  VectorParamsAs1DForOutWhenUnconnected=off
  wires:
  n/1 -> FIMWB_063/1(Original)
  FIMWB_063/1(Result) -> a/1

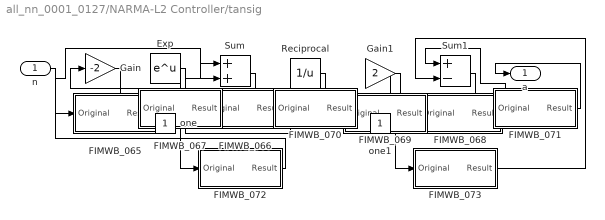
== system all_nn_0001_0127/NARMA-L2 Controller/tansig ==
  n : Inport
  Exp : Math  SignedPower=on
  FIMWB_065 : Subsystem  Tag=fimwb.fault.65
  FIMWB_066 : Subsystem  Tag=fimwb.fault.66
  FIMWB_067 : Subsystem  Tag=fimwb.fault.67
  FIMWB_068 : Subsystem  Tag=fimwb.fault.68
  FIMWB_069 : Subsystem  Tag=fimwb.fault.69
  FIMWB_070 : Subsystem  Tag=fimwb.fault.70
  FIMWB_071 : Subsystem  Tag=fimwb.fault.71
  FIMWB_072 : Subsystem  Tag=fimwb.fault.72
  FIMWB_073 : Subsystem  Tag=fimwb.fault.73
  Gain : Gain  Gain=-2  SaturateOnIntegerOverflow=on  OutDataTypeStr=Inherit: Same as input  ParamDataTypeStr=Inherit: Same as input
  Gain1 : Gain  Gain=2  SaturateOnIntegerOverflow=on  OutDataTypeStr=Inherit: Same as input  ParamDataTypeStr=Inherit: Same as input
  Reciprocal : Math  Operator=reciprocal  SignedPower=on
  Sum : Sum  InputSameDT=on  SaturateOnIntegerOverflow=on  OutDataTypeStr=Inherit: Same as first input
  Sum1 : Sum  Inputs=+-  InputSameDT=on  SaturateOnIntegerOverflow=on  OutDataTypeStr=Inherit: Same as first input
  one : Constant
  one1 : Constant
  a : Outport  VectorParamsAs1DForOutWhenUnconnected=off
  wires:
  n/1 -> FIMWB_065/1(Original)
  FIMWB_065/1(Result) -> Gain/1
  Exp/1 -> FIMWB_066/1(Original)
  FIMWB_066/1(Result) -> Sum/1
  Gain/1 -> FIMWB_067/1(Original)
  FIMWB_067/1(Result) -> Exp/1
  Gain1/1 -> FIMWB_068/1(Original)
  FIMWB_068/1(Result) -> Sum1/1
  Reciprocal/1 -> FIMWB_069/1(Original)
  FIMWB_069/1(Result) -> Gain1/1
  Sum/1 -> FIMWB_070/1(Original)
  FIMWB_070/1(Result) -> Reciprocal/1
  Sum1/1 -> FIMWB_071/1(Original)
  FIMWB_071/1(Result) -> a/1
  one/1 -> FIMWB_072/1(Original)
  FIMWB_072/1(Result) -> Sum/2
  one1/1 -> FIMWB_073/1(Original)
  FIMWB_073/1(Result) -> Sum1/2

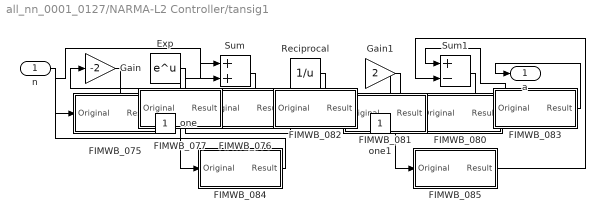
== system all_nn_0001_0127/NARMA-L2 Controller/tansig1 ==
  n : Inport
  Exp : Math  SignedPower=on
  FIMWB_075 : Subsystem  Tag=fimwb.fault.75
  FIMWB_076 : Subsystem  Tag=fimwb.fault.76
  FIMWB_077 : Subsystem  Tag=fimwb.fault.77
  FIMWB_080 : Subsystem  Tag=fimwb.fault.80
  FIMWB_081 : Subsystem  Tag=fimwb.fault.81
  FIMWB_082 : Subsystem  Tag=fimwb.fault.82
  FIMWB_083 : Subsystem  Tag=fimwb.fault.83
  FIMWB_084 : Subsystem  Tag=fimwb.fault.84
  FIMWB_085 : Subsystem  Tag=fimwb.fault.85
  Gain : Gain  Gain=-2  SaturateOnIntegerOverflow=on  OutDataTypeStr=Inherit: Same as input  ParamDataTypeStr=Inherit: Same as input
  Gain1 : Gain  Gain=2  SaturateOnIntegerOverflow=on  OutDataTypeStr=Inherit: Same as input  ParamDataTypeStr=Inherit: Same as input
  Reciprocal : Math  Operator=reciprocal  SignedPower=on
  Sum : Sum  InputSameDT=on  SaturateOnIntegerOverflow=on  OutDataTypeStr=Inherit: Same as first input
  Sum1 : Sum  Inputs=+-  InputSameDT=on  SaturateOnIntegerOverflow=on  OutDataTypeStr=Inherit: Same as first input
  one : Constant
  one1 : Constant
  a : Outport  VectorParamsAs1DForOutWhenUnconnected=off
  wires:
  n/1 -> FIMWB_075/1(Original)
  FIMWB_075/1(Result) -> Gain/1
  Exp/1 -> FIMWB_076/1(Original)
  FIMWB_076/1(Result) -> Sum/1
  Gain/1 -> FIMWB_077/1(Original)
  FIMWB_077/1(Result) -> Exp/1
  Gain1/1 -> FIMWB_080/1(Original)
  FIMWB_080/1(Result) -> Sum1/1
  Reciprocal/1 -> FIMWB_081/1(Original)
  FIMWB_081/1(Result) -> Gain1/1
  Sum/1 -> FIMWB_082/1(Original)
  FIMWB_082/1(Result) -> Reciprocal/1
  Sum1/1 -> FIMWB_083/1(Original)
  FIMWB_083/1(Result) -> a/1
  one/1 -> FIMWB_084/1(Original)
  FIMWB_084/1(Result) -> Sum/2
  one1/1 -> FIMWB_085/1(Original)
  FIMWB_085/1(Result) -> Sum1/2

== system all_nn_0001_0127/Plant (Magnet Levitation)/FIMWB_001 ==
  Original : Inport
  Result : Outport
  wires:
  Original/1 -> Result/1

== system all_nn_0001_0127/Plant (Magnet Levitation)/FIMWB_002 ==
  Original : Inport
  Result : Outport
  wires:
  Original/1 -> Result/1

== system all_nn_0001_0127/Plant (Magnet Levitation)/FIMWB_003 ==
  Original : Inport
  Result : Outport
  wires:
  Original/1 -> Result/1

== system all_nn_0001_0127/Plant (Magnet Levitation)/FIMWB_088 ==
  Original : Inport
  Result : Outport
  wires:
  Original/1 -> Result/1

== system all_nn_0001_0127/Plant (Magnet Levitation)/FIMWB_089 ==
  Original : Inport
  Result : Outport
  wires:
  Original/1 -> Result/1

== system all_nn_0001_0127/Plant (Magnet Levitation)/FIMWB_092 ==
  Original : Inport
  Result : Outport
  wires:
  Original/1 -> Result/1

== system all_nn_0001_0127/Plant (Magnet Levitation)/FIMWB_093 ==
  Original : Inport
  Result : Outport
  wires:
  Original/1 -> Result/1

== system all_nn_0001_0127/Plant (Magnet Levitation)/FIMWB_094 ==
  Original : Inport
  Result : Outport
  wires:
  Original/1 -> Result/1

== system all_nn_0001_0127/Plant (Magnet Levitation)/FIMWB_095 ==
  Original : Inport
  Result : Outport
  wires:
  Original/1 -> Result/1

== system all_nn_0001_0127/Plant (Magnet Levitation)/FIMWB_096 ==
  Original : Inport
  Result : Outport
  wires:
  Original/1 -> Result/1

== system all_nn_0001_0127/Plant (Magnet Levitation)/FIMWB_097 ==
  Original : Inport
  Result : Outport
  wires:
  Original/1 -> Result/1

== system all_nn_0001_0127/Plant (Magnet Levitation)/FIMWB_098 ==
  Original : Inport
  Result : Outport
  wires:
  Original/1 -> Result/1

== system all_nn_0001_0127/Plant (Magnet Levitation)/FIMWB_099 ==
  Original : Inport
  Result : Outport
  wires:
  Original/1 -> Result/1

== system all_nn_0001_0127/Plant (Magnet Levitation)/FIMWB_100 ==
  Original : Inport
  Result : Outport
  wires:
  Original/1 -> Result/1

== system all_nn_0001_0127/Plant (Magnet Levitation)/FIMWB_101 ==
  Original : Inport
  Result : Outport
  wires:
  Original/1 -> Result/1

== system all_nn_0001_0127/Plant (Magnet Levitation)/FIMWB_102 ==
  Original : Inport
  Result : Outport
  wires:
  Original/1 -> Result/1

== system all_nn_0001_0127/Plant (Magnet Levitation)/FIMWB_103 ==
  Original : Inport
  Result : Outport
  wires:
  Original/1 -> Result/1

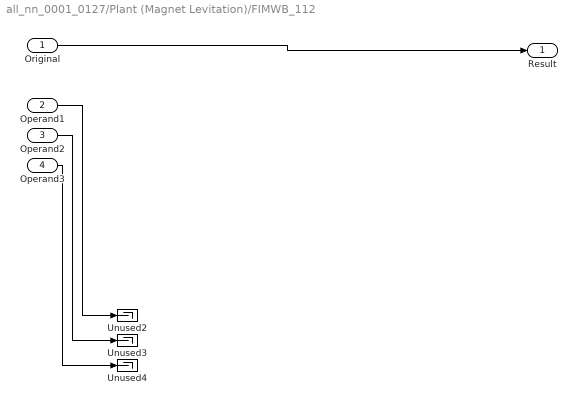
== system all_nn_0001_0127/Plant (Magnet Levitation)/FIMWB_112 ==
  Original : Inport
  Operand1 : Inport  Port=2
  Operand2 : Inport  Port=3
  Operand3 : Inport  Port=4
  Unused2 : Terminator
  Unused3 : Terminator
  Unused4 : Terminator
  Result : Outport
  wires:
  Original/1 -> Result/1
  Operand1/1 -> Unused2/1
  Operand2/1 -> Unused3/1
  Operand3/1 -> Unused4/1

== system all_nn_0001_0127/Plant (Magnet Levitation)/FIMWB_113 ==
  Original : Inport
  Operand1 : Inport  Port=2
  Operand2 : Inport  Port=3
  Unused2 : Terminator
  Unused3 : Terminator
  Result : Outport
  wires:
  Original/1 -> Result/1
  Operand1/1 -> Unused2/1
  Operand2/1 -> Unused3/1

== system all_nn_0001_0127/Plant (Magnet Levitation)/FIMWB_114 ==
  Original : Inport
  Operand1 : Inport  Port=2
  Operand2 : Inport  Port=3
  Unused2 : Terminator
  Unused3 : Terminator
  Result : Outport
  wires:
  Original/1 -> Result/1
  Operand1/1 -> Unused2/1
  Operand2/1 -> Unused3/1

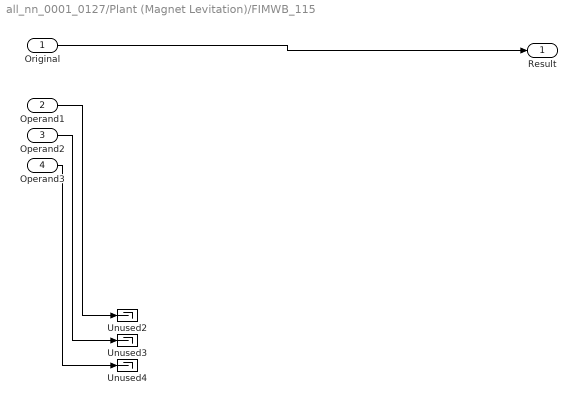
== system all_nn_0001_0127/Plant (Magnet Levitation)/FIMWB_115 ==
  Original : Inport
  Operand1 : Inport  Port=2
  Operand2 : Inport  Port=3
  Operand3 : Inport  Port=4
  Unused2 : Terminator
  Unused3 : Terminator
  Unused4 : Terminator
  Result : Outport
  wires:
  Original/1 -> Result/1
  Operand1/1 -> Unused2/1
  Operand2/1 -> Unused3/1
  Operand3/1 -> Unused4/1

== system all_nn_0001_0127/Plant (Magnet Levitation)/FIMWB_116 ==
  Original : Inport
  Result : Outport
  wires:
  Original/1 -> Result/1

== system all_nn_0001_0127/Plant (Magnet Levitation)/FIMWB_123 ==
  Original : Inport
  Result : Outport
  wires:
  Original/1 -> Result/1

== system all_nn_0001_0127/Plant (Magnet Levitation)/FIMWB_125 ==
  Original : Inport
  Result : Outport
  wires:
  Original/1 -> Result/1

== system all_nn_0001_0127/Plant (Magnet Levitation)/FIMWB_126 ==
  Original : Inport
  Result : Outport
  wires:
  Original/1 -> Result/1

== system all_nn_0001_0127/NARMA-L2 Controller/netsum/FIMWB_045 ==
  Original : Inport
  Result : Outport
  wires:
  Original/1 -> Result/1

== system all_nn_0001_0127/NARMA-L2 Controller/netsum/FIMWB_046 ==
  Original : Inport
  Result : Outport
  wires:
  Original/1 -> Result/1

== system all_nn_0001_0127/NARMA-L2 Controller/netsum/FIMWB_047 ==
  Original : Inport
  Result : Outport
  wires:
  Original/1 -> Result/1

== system all_nn_0001_0127/NARMA-L2 Controller/netsum1/FIMWB_049 ==
  Original : Inport
  Result : Outport
  wires:
  Original/1 -> Result/1

== system all_nn_0001_0127/NARMA-L2 Controller/netsum1/FIMWB_050 ==
  Original : Inport
  Result : Outport
  wires:
  Original/1 -> Result/1

== system all_nn_0001_0127/NARMA-L2 Controller/netsum1/FIMWB_051 ==
  Original : Inport
  Result : Outport
  wires:
  Original/1 -> Result/1

== system all_nn_0001_0127/NARMA-L2 Controller/netsum1/FIMWB_110 ==
  Original : Inport
  Operand1 : Inport  Port=2
  Operand2 : Inport  Port=3
  Unused2 : Terminator
  Unused3 : Terminator
  Result : Outport
  wires:
  Original/1 -> Result/1
  Operand1/1 -> Unused2/1
  Operand2/1 -> Unused3/1

== system all_nn_0001_0127/NARMA-L2 Controller/netsum2/FIMWB_053 ==
  Original : Inport
  Result : Outport
  wires:
  Original/1 -> Result/1

== system all_nn_0001_0127/NARMA-L2 Controller/netsum2/FIMWB_054 ==
  Original : Inport
  Result : Outport
  wires:
  Original/1 -> Result/1

== system all_nn_0001_0127/NARMA-L2 Controller/netsum2/FIMWB_055 ==
  Original : Inport
  Result : Outport
  wires:
  Original/1 -> Result/1

== system all_nn_0001_0127/NARMA-L2 Controller/netsum3/FIMWB_057 ==
  Original : Inport
  Result : Outport
  wires:
  Original/1 -> Result/1

== system all_nn_0001_0127/NARMA-L2 Controller/netsum3/FIMWB_058 ==
  Original : Inport
  Result : Outport
  wires:
  Original/1 -> Result/1

== system all_nn_0001_0127/NARMA-L2 Controller/netsum3/FIMWB_059 ==
  Original : Inport
  Result : Outport
  wires:
  Original/1 -> Result/1

== system all_nn_0001_0127/NARMA-L2 Controller/netsum3/FIMWB_111 ==
  Original : Inport
  Operand1 : Inport  Port=2
  Operand2 : Inport  Port=3
  Unused2 : Terminator
  Unused3 : Terminator
  Result : Outport
  wires:
  Original/1 -> Result/1
  Operand1/1 -> Unused2/1
  Operand2/1 -> Unused3/1

== system all_nn_0001_0127/NARMA-L2 Controller/purelin/FIMWB_061 ==
  Original : Inport
  Result : Outport
  wires:
  Original/1 -> Result/1

== system all_nn_0001_0127/NARMA-L2 Controller/purelin1/FIMWB_063 ==
  Original : Inport
  Result : Outport
  wires:
  Original/1 -> Result/1

== system all_nn_0001_0127/NARMA-L2 Controller/tansig/FIMWB_065 ==
  Original : Inport
  Result : Outport
  wires:
  Original/1 -> Result/1

== system all_nn_0001_0127/NARMA-L2 Controller/tansig/FIMWB_066 ==
  Original : Inport
  Result : Outport
  wires:
  Original/1 -> Result/1

== system all_nn_0001_0127/NARMA-L2 Controller/tansig/FIMWB_067 ==
  Original : Inport
  Result : Outport
  wires:
  Original/1 -> Result/1

== system all_nn_0001_0127/NARMA-L2 Controller/tansig/FIMWB_068 ==
  Original : Inport
  Result : Outport
  wires:
  Original/1 -> Result/1

== system all_nn_0001_0127/NARMA-L2 Controller/tansig/FIMWB_069 ==
  Original : Inport
  Result : Outport
  wires:
  Original/1 -> Result/1

== system all_nn_0001_0127/NARMA-L2 Controller/tansig/FIMWB_070 ==
  Original : Inport
  Result : Outport
  wires:
  Original/1 -> Result/1

== system all_nn_0001_0127/NARMA-L2 Controller/tansig/FIMWB_071 ==
  Original : Inport
  Result : Outport
  wires:
  Original/1 -> Result/1

== system all_nn_0001_0127/NARMA-L2 Controller/tansig/FIMWB_072 ==
  Original : Inport
  Result : Outport
  wires:
  Original/1 -> Result/1

== system all_nn_0001_0127/NARMA-L2 Controller/tansig/FIMWB_073 ==
  Original : Inport
  Result : Outport
  wires:
  Original/1 -> Result/1

== system all_nn_0001_0127/NARMA-L2 Controller/tansig1/FIMWB_075 ==
  Original : Inport
  Result : Outport
  wires:
  Original/1 -> Result/1

== system all_nn_0001_0127/NARMA-L2 Controller/tansig1/FIMWB_076 ==
  Original : Inport
  Result : Outport
  wires:
  Original/1 -> Result/1

== system all_nn_0001_0127/NARMA-L2 Controller/tansig1/FIMWB_077 ==
  Original : Inport
  Result : Outport
  wires:
  Original/1 -> Result/1

== system all_nn_0001_0127/NARMA-L2 Controller/tansig1/FIMWB_080 ==
  Original : Inport
  Result : Outport
  wires:
  Original/1 -> Result/1

== system all_nn_0001_0127/NARMA-L2 Controller/tansig1/FIMWB_081 ==
  Original : Inport
  Result : Outport
  wires:
  Original/1 -> Result/1

== system all_nn_0001_0127/NARMA-L2 Controller/tansig1/FIMWB_082 ==
  Original : Inport
  Result : Outport
  wires:
  Original/1 -> Result/1

== system all_nn_0001_0127/NARMA-L2 Controller/tansig1/FIMWB_083 ==
  Original : Inport
  Result : Outport
  wires:
  Original/1 -> Result/1

== system all_nn_0001_0127/NARMA-L2 Controller/tansig1/FIMWB_084 ==
  Original : Inport
  Result : Outport
  wires:
  Original/1 -> Result/1

== system all_nn_0001_0127/NARMA-L2 Controller/tansig1/FIMWB_085 ==
  Original : Inport
  Result : Outport
  wires:
  Original/1 -> Result/1
